simulink model "NBMS_ChargeOCV"  (R2026b)
settings: Solver=FixedStepDiscrete  StopTime=20  FixedStep=0.1
undefined symbols (not defined in the file): X_SOC_VS_OCV_CHG, Y_SOC_VS_OCV_CHG
settings Model: Creator=hp  LastModifiedBy=rathi
settings OptimizationCC: DefaultParameterBehavior=Inlined  DifferentSizesBufferReuse=on  EfficientTunableParamExpr=on  EnhancedBackFolding=on  OptimizationCustomize=off  OptimizeBlockOrder=speed  PassReuseOutputArgsAs=Individual arguments  RemoveInternalMemoryZeroInit=on  RemoveRootLevelIOMemoryZeroInit=on
settings DebuggingCC: ParameterTunabilityLossMsg=error
settings SFSimCC: MATLABDynamicMemAlloc=off
settings RTWCC: Description=Embedded Coder  GenCodeOnly=on  PackageGeneratedCodeAndArtifacts=on  SystemTargetFile=ert.tlc  TemplateMakefile=ert_default_tmf
settings CodeAppCC: ForceParamTrailComments=on  IgnoreCustomStorageClasses=off  InsertBlockDesc=on  OperatorAnnotations=on  SFDataObjDesc=on  SimulinkDataObjDesc=on
settings ERTTargetCC: DynamicArrayContainerType=coder::array  GenerateSampleERTMain=on
settings ConfigComp: DVDefectChecker=on  DVDetectOutOfBounds=on  DVHarnessSource=Signal Editor  DVModelReferenceHarness=on  DVTestSuiteOptimization=Auto

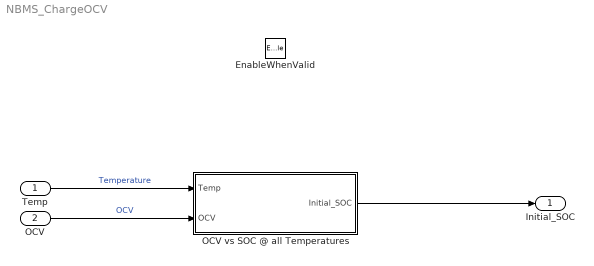
== system NBMS_ChargeOCV ==
  Temp : Inport  OutDataTypeStr=double
  OCV : Inport  Port=2  OutDataTypeStr=fixdt(1,16,0.001,0)
  EnableWhenValid : EnablePort  StatesWhenEnabling=reset  OutDataTypeStr=boolean
  OCV vs SOC @ all Temperatures : Subsystem  TreatAsAtomicUnit=on
  Initial_SOC : Outport  OutputWhenDisabled=reset  InitialOutput=0
  wires:
  Temp/1 -> OCV vs SOC @ all Temperatures/1(Temp)  "Temperature"
  OCV vs SOC @ all Temperatures/1(Initial_SOC) -> Initial_SOC/1
  OCV/1 -> OCV vs SOC @ all Temperatures/2(OCV)  "OCV"

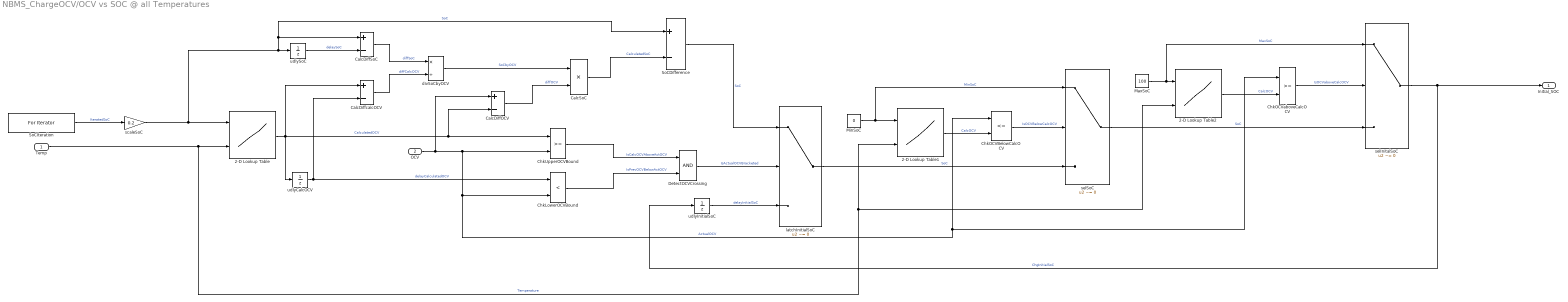
== system NBMS_ChargeOCV/OCV vs SOC @ all Temperatures ==
  Temp : Inport  OutDataTypeStr=double
  OCV : Inport  Port=2  OutDataTypeStr=fixdt(1,16,0.001,0)
  2-D Lookup Table : Lookup_n-D  BreakpointsForDimension1=X_SOC_VS_OCV_CHG  BreakpointsForDimension2=Y_SOC_VS_OCV_CHG  Table=[2.9340000000000002 2.9289999999999998 2.9199999999999999 2.8999999999999999 2.911 2.903 2.9220000000000002;3.2599999999999998 3.274 3.2709999999999999 3.2709999999999999 3.254 3.238 3.2400000000000002;3.387 3.399 3.3969999999999998 3.3969999999999998 3.3849999999999998 3.3620000000000001 3.363;3.4359999999999999 3.4420000000000002 3.4420000000000002 3.4409999999999998 3.4390000000000001 3.4289999999999998 3.4300000000000002;3.4809999999999999 3.4910000000000001 3.4910000000000001 3.4929999999999999 3.492 3.4790000000000001 3.4809999999999999;3.5379999999999998 3.5470000000000002 3.5459999999999998 3.5470000000000002 3.54 3.5339999999999998 3.5339999999999998;3.5859999999999999 3.5920000000000001 3.5920000000000001 3.593 3.589 3.5819999999999999 3.5819999999999999;3.6160000000000001 3.621 3.6219999999999999 3.6240000000000001 3.6219999999999999 3.6219999999999999 3.6230000000000002;3.6440000000000001 3.6499999999999999 3.6509999999999998 3.653 3.6520000000000001 3.653 3.6560000000000001;3.677 3.6829999999999998 3.6850000000000001 3.6869999999999998 3.6859999999999999 3.6880000000000002 3.6909999999999998;3.7189999999999999 3.726 3.7269999999999999 3.73 3.7280000000000002 3.7309999999999999 3.734;3.766 3.7719999999999998 3.774 3.7770000000000001 3.7759999999999998 3.7770000000000001 3.7799999999999998;3.819 3.8370000000000002 3.8380000000000001 3.8399999999999999 3.835 3.8290000000000002 3.831;3.8799999999999999 3.8860000000000001 3.8860000000000001 3.887 3.8849999999999998 3.883 3.8820000000000001;3.9129999999999998 3.9180000000000001 3.919 3.9199999999999999 3.9180000000000001 3.9169999999999998 3.9169999999999998;3.952 3.9580000000000002 3.9590000000000001 3.96 3.9580000000000002 3.9580000000000002 3.9580000000000002;4.0099999999999998 4.0170000000000003 4.0170000000000003 4.0190000000000001 4.0170000000000003 4.016 4.016;4.0609999999999999 4.0659999999999998 4.0670000000000002 4.0679999999999996 4.0670000000000002 4.0670000000000002 4.0670000000000002;4.0759999999999996 4.0800000000000001 4.0819999999999999 4.0830000000000002 4.0830000000000002 4.0830000000000002 4.0839999999999996;4.0899999999999999 4.0960000000000001 4.0979999999999999 4.0999999999999996 4.0990000000000002 4.0979999999999999 4.0990000000000002;4.1849999999999996 4.1849999999999996 4.1849999999999996 4.1849999999999996 4.1849999999999996 4.1849999999999996 4.1849999999999996]  InternalRulePriority=Speed  RndMeth=Simplest
      settings: InputPortMap=u0,u1
  2-D Lookup Table1 : Lookup_n-D  BreakpointsForDimension1=X_SOC_VS_OCV_CHG  BreakpointsForDimension2=Y_SOC_VS_OCV_CHG  Table=[2.9340000000000002 2.9289999999999998 2.9199999999999999 2.8999999999999999 2.911 2.903 2.9220000000000002;3.2599999999999998 3.274 3.2709999999999999 3.2709999999999999 3.254 3.238 3.2400000000000002;3.387 3.399 3.3969999999999998 3.3969999999999998 3.3849999999999998 3.3620000000000001 3.363;3.4359999999999999 3.4420000000000002 3.4420000000000002 3.4409999999999998 3.4390000000000001 3.4289999999999998 3.4300000000000002;3.4809999999999999 3.4910000000000001 3.4910000000000001 3.4929999999999999 3.492 3.4790000000000001 3.4809999999999999;3.5379999999999998 3.5470000000000002 3.5459999999999998 3.5470000000000002 3.54 3.5339999999999998 3.5339999999999998;3.5859999999999999 3.5920000000000001 3.5920000000000001 3.593 3.589 3.5819999999999999 3.5819999999999999;3.6160000000000001 3.621 3.6219999999999999 3.6240000000000001 3.6219999999999999 3.6219999999999999 3.6230000000000002;3.6440000000000001 3.6499999999999999 3.6509999999999998 3.653 3.6520000000000001 3.653 3.6560000000000001;3.677 3.6829999999999998 3.6850000000000001 3.6869999999999998 3.6859999999999999 3.6880000000000002 3.6909999999999998;3.7189999999999999 3.726 3.7269999999999999 3.73 3.7280000000000002 3.7309999999999999 3.734;3.766 3.7719999999999998 3.774 3.7770000000000001 3.7759999999999998 3.7770000000000001 3.7799999999999998;3.819 3.8370000000000002 3.8380000000000001 3.8399999999999999 3.835 3.8290000000000002 3.831;3.8799999999999999 3.8860000000000001 3.8860000000000001 3.887 3.8849999999999998 3.883 3.8820000000000001;3.9129999999999998 3.9180000000000001 3.919 3.9199999999999999 3.9180000000000001 3.9169999999999998 3.9169999999999998;3.952 3.9580000000000002 3.9590000000000001 3.96 3.9580000000000002 3.9580000000000002 3.9580000000000002;4.0099999999999998 4.0170000000000003 4.0170000000000003 4.0190000000000001 4.0170000000000003 4.016 4.016;4.0609999999999999 4.0659999999999998 4.0670000000000002 4.0679999999999996 4.0670000000000002 4.0670000000000002 4.0670000000000002;4.0759999999999996 4.0800000000000001 4.0819999999999999 4.0830000000000002 4.0830000000000002 4.0830000000000002 4.0839999999999996;4.0899999999999999 4.0960000000000001 4.0979999999999999 4.0999999999999996 4.0990000000000002 4.0979999999999999 4.0990000000000002;4.1849999999999996 4.1849999999999996 4.1849999999999996 4.1849999999999996 4.1849999999999996 4.1849999999999996 4.1849999999999996]  InternalRulePriority=Speed  RndMeth=Simplest
      settings: InputPortMap=u0,u1
  2-D Lookup Table2 : Lookup_n-D  BreakpointsForDimension1=X_SOC_VS_OCV_CHG  BreakpointsForDimension2=Y_SOC_VS_OCV_CHG  Table=[2.9340000000000002 2.9289999999999998 2.9199999999999999 2.8999999999999999 2.911 2.903 2.9220000000000002;3.2599999999999998 3.274 3.2709999999999999 3.2709999999999999 3.254 3.238 3.2400000000000002;3.387 3.399 3.3969999999999998 3.3969999999999998 3.3849999999999998 3.3620000000000001 3.363;3.4359999999999999 3.4420000000000002 3.4420000000000002 3.4409999999999998 3.4390000000000001 3.4289999999999998 3.4300000000000002;3.4809999999999999 3.4910000000000001 3.4910000000000001 3.4929999999999999 3.492 3.4790000000000001 3.4809999999999999;3.5379999999999998 3.5470000000000002 3.5459999999999998 3.5470000000000002 3.54 3.5339999999999998 3.5339999999999998;3.5859999999999999 3.5920000000000001 3.5920000000000001 3.593 3.589 3.5819999999999999 3.5819999999999999;3.6160000000000001 3.621 3.6219999999999999 3.6240000000000001 3.6219999999999999 3.6219999999999999 3.6230000000000002;3.6440000000000001 3.6499999999999999 3.6509999999999998 3.653 3.6520000000000001 3.653 3.6560000000000001;3.677 3.6829999999999998 3.6850000000000001 3.6869999999999998 3.6859999999999999 3.6880000000000002 3.6909999999999998;3.7189999999999999 3.726 3.7269999999999999 3.73 3.7280000000000002 3.7309999999999999 3.734;3.766 3.7719999999999998 3.774 3.7770000000000001 3.7759999999999998 3.7770000000000001 3.7799999999999998;3.819 3.8370000000000002 3.8380000000000001 3.8399999999999999 3.835 3.8290000000000002 3.831;3.8799999999999999 3.8860000000000001 3.8860000000000001 3.887 3.8849999999999998 3.883 3.8820000000000001;3.9129999999999998 3.9180000000000001 3.919 3.9199999999999999 3.9180000000000001 3.9169999999999998 3.9169999999999998;3.952 3.9580000000000002 3.9590000000000001 3.96 3.9580000000000002 3.9580000000000002 3.9580000000000002;4.0099999999999998 4.0170000000000003 4.0170000000000003 4.0190000000000001 4.0170000000000003 4.016 4.016;4.0609999999999999 4.0659999999999998 4.0670000000000002 4.0679999999999996 4.0670000000000002 4.0670000000000002 4.0670000000000002;4.0759999999999996 4.0800000000000001 4.0819999999999999 4.0830000000000002 4.0830000000000002 4.0830000000000002 4.0839999999999996;4.0899999999999999 4.0960000000000001 4.0979999999999999 4.0999999999999996 4.0990000000000002 4.0979999999999999 4.0990000000000002;4.1849999999999996 4.1849999999999996 4.1849999999999996 4.1849999999999996 4.1849999999999996 4.1849999999999996 4.1849999999999996]  InternalRulePriority=Speed  RndMeth=Simplest
      settings: InputPortMap=u0,u1
  CalcDiffOCV : Sum  Inputs=+-
  CalcDiffSoC : Sum  Inputs=+-
  CalcDiffcalcOCV : Sum  Inputs=+-
  CalcSoC : Product
  ChkLowerOCVBound : RelationalOperator  Operator=<  OutDataTypeStr=boolean  RndMeth=Simplest  InputSameDT=off
  ChkOCVBelowCalcOCV : RelationalOperator  Operator=<=  OutDataTypeStr=boolean  RndMeth=Simplest  InputSameDT=off
  ChkOCVaboveCalcOCV : RelationalOperator  OutDataTypeStr=boolean  RndMeth=Simplest  InputSameDT=off
  ChkUpperOCVBound : RelationalOperator  OutDataTypeStr=boolean  RndMeth=Simplest  InputSameDT=off
  "DetectOCVCrossing " : Logic  AllPortsSameDT=off  OutDataTypeStr=boolean
  MaxSoC : Constant  Value=100
  MinSoC : Constant  Value=0
  SoCDifference : Sum  Inputs=+-
  SoCIteration : ForIterator  ResetStates=reset  IterationLimit=501  IndexMode=Zero-based  IterationVariableDataType=double
  divSoCbyOCV : Product  Inputs=*/
  latchInitialSoC : Switch  Criteria=u2 ~= 0  SaturateOnIntegerOverflow=off  InputSameDT=off
  scaleSoC : Gain  Gain=0.2
  selInitalSoC : Switch  Criteria=u2 ~= 0  SaturateOnIntegerOverflow=off  InputSameDT=off
  selSoC : Switch  Criteria=u2 ~= 0  SaturateOnIntegerOverflow=off  InputSameDT=off
  udlyCalcOCV : UnitDelay  SampleTime=-1
  udlyInitialSoC : UnitDelay  SampleTime=-1
  udlySoC : UnitDelay  SampleTime=-1
  Initial_SOC : Outport
  wires:
  Temp/1 -> 2-D Lookup Table2/2, 2-D Lookup Table1/2, 2-D Lookup Table/2  "Temperature"
  latchInitialSoC/1 -> selSoC/3  "SoC"
  2-D Lookup Table/1 -> ChkUpperOCVBound/1, CalcDiffOCV/2, CalcDiffcalcOCV/1, udlyCalcOCV/1  "CalculatedOCV"
  OCV/1 -> ChkLowerOCVBound/2, ChkOCVBelowCalcOCV/1, ChkOCVaboveCalcOCV/1, ChkUpperOCVBound/2, CalcDiffOCV/1  "ActualOCV"
  ChkOCVBelowCalcOCV/1 -> selSoC/2  "IsOCVBelowCalcOCV"
  udlyInitialSoC/1 -> latchInitialSoC/3  "delayInitialSoC"
  CalcDiffcalcOCV/1 -> divSoCbyOCV/2  "diffCalcOCV"
  selSoC/1 -> selInitalSoC/3  "SoC"
  MinSoC/1 -> selSoC/1, 2-D Lookup Table1/1  "MinSoC"
  SoCDifference/1 -> latchInitialSoC/1  "SoC"
  udlyCalcOCV/1 -> ChkLowerOCVBound/1, CalcDiffcalcOCV/2  "delayCalculatedOCV"
  ChkOCVaboveCalcOCV/1 -> selInitalSoC/2  "IsOCVaboveCalcOCV"
  divSoCbyOCV/1 -> CalcSoC/1  "SoCbyOCV"
  selInitalSoC/1 -> udlyInitialSoC/1, Initial_SOC/1  "ChgInitialSoC"
  CalcDiffOCV/1 -> CalcSoC/2  "diffOCV"
  SoCIteration/1 -> scaleSoC/1  "IteratedSoC"
  CalcSoC/1 -> SoCDifference/2  "CalculatedSoC"
  MaxSoC/1 -> selInitalSoC/1, 2-D Lookup Table2/1  "MaxSoC"
  scaleSoC/1 -> 2-D Lookup Table/1, SoCDifference/1, CalcDiffSoC/1, udlySoC/1  "SoC"
  "DetectOCVCrossing "/1 -> latchInitialSoC/2  "IsActualOCVBracketed"
  CalcDiffSoC/1 -> divSoCbyOCV/1  "diffSoC"
  udlySoC/1 -> CalcDiffSoC/2  "delaySoC"
  ChkUpperOCVBound/1 -> "DetectOCVCrossing "/1  "IsCalcOCVAboveActOCV"
  ChkLowerOCVBound/1 -> "DetectOCVCrossing "/2  "IsPrevOCVBelowActOCV"
  2-D Lookup Table1/1 -> ChkOCVBelowCalcOCV/2  "CalcOCV"
  2-D Lookup Table2/1 -> ChkOCVaboveCalcOCV/2  "CalcOCV"
